simulink model "aerodynamic_model_V1_2_Wrench"  (R2025b)
settings: Solver=ode4  StartTime=0.0  StopTime=0.3  FixedStep=Ts  RelTol=1e-3
InitFcn:
  | % Run initial_main.m first to load Ad,As,Tq_prop,Tq_mass,...
values from neighbouring files (symbols this model uses):
  alpha_du0_v_tail_L = trim_aero_ic.v_tail_L.alpha_du0    [initial_main_V1_1.m]
  alpha_du0_v_tail_R = trim_aero_ic.v_tail_R.alpha_du0    [initial_main_V1_1.m]
  alpha_du0_wing_L = trim_aero_ic.wing_L.alpha_du0    [initial_main_V1_1.m]
  alpha_du0_wing_R = trim_aero_ic.wing_R.alpha_du0    [initial_main_V1_1.m]
  As = sys_sd.A    [initial_main_V1_1.m]
  BladePitch_deg = 34    [initial_main_V1_1.m]
  Bs = sys_sd.B    [initial_main_V1_1.m]
  Cs = sys_sd.C    [initial_main_V1_1.m]
  ctrl_delta_lim_deg = strips.delta_lim_deg    [initial_main_V1_1.m]
  ctrl_map_aileron_L = aero.wing_L.map_aileron(:)    [initial_main_V1_1.m]
  ctrl_map_aileron_R = aero.wing_R.map_aileron(:)    [initial_main_V1_1.m]
  ctrl_map_tail_L = aero.v_tail_L.map_tail(:)    [initial_main_V1_1.m]
  ctrl_map_tail_R = aero.v_tail_R.map_tail(:)    [initial_main_V1_1.m]
  Ds = sys_sd.D    [initial_main_V1_1.m]
  I_cg_b = R_sb * I_cg_m * R_sb.'    [aeroelastic.m]    (also in initial_main_V1_1.m = grav.I_cg_b)
  I_cg_b_inv = R_sb * I_cg_m_inv * R_sb.'    [aeroelastic.m]    (also in initial_main_V1_1.m = grav.I_cg_b_inv)
  m_node = zeros(n_id, 1)    [aeroelastic.m]    (also in generate_pullup_load_cloud.m = evalin('base', 'm_node(:)'); initial_main_V1_1.m = nodal.m_node)
  m_total_kg = evalin('base', 'm_total_kg')    [generate_pullup_load_cloud.m]    (also in initial_main_V1_1.m = grav.m_total_kg)
  n_modes = size(Phi, 2)    [aeroelastic.m]    (also in initial_main_V1_1.m = n_rigid + n_elastic)
  ones_1_tail = ones(1, size(r_cg2ac_b_v_tail_L, 2))    [initial_main_V1_1.m]
  ones_1_wing = ones(1, size(r_cg2ac_b_wing_L, 2))    [initial_main_V1_1.m]
  Phi = evalin('base', 'Phi')    [generate_pullup_load_cloud.m]    (also in initial_main_V1_1.m = strips.Phi)
  polar_alpha_deg = polar.alpha_deg(:).'    [initial_main_V1_1.m]
  polar_CD = polar.CD(:).'    [initial_main_V1_1.m]
  polar_CDp = polar.CDp(:).'    [initial_main_V1_1.m]
  polar_CL = polar.CL(:).'    [initial_main_V1_1.m]
  polar_CM = polar.CM(:).'    [initial_main_V1_1.m]
  r_cg2ac_b_v_tail_L = R_sb * aero.v_tail_L.r_ac_s    [initial_main_V1_1.m]
  r_cg2ac_b_v_tail_R = R_sb * aero.v_tail_R.r_ac_s    [initial_main_V1_1.m]
  r_cg2ac_b_wing_L = R_sb * aero.wing_L.r_ac_s    [initial_main_V1_1.m]
  r_cg2ac_b_wing_R = R_sb * aero.wing_R.r_ac_s    [initial_main_V1_1.m]
  r_cg2kink_b = eng.r_cg2kink_b    [initial_main_V1_1.m]
  r_cg2node_b = aeroelastic.node_arms(nodes, 'R_sb', R_sb).r_cg2node_b    [initial_main_V1_1.m]
  surface_nodes = aeroelastic.surface_load_nodes(nodes)    [initial_main_V1_1.m]
  T_aero2W = aeroelastic.wing_aileron_to_W(strips).T    [initial_main_V1_1.m]
  T_prop2W = load_maps.T_prop2W    [initial_main_V1_1.m]
  Tq_mass = load_maps.Tq_mass    [initial_main_V1_1.m]
  trim_Attitude_rad0 = trim_default.Attitude_rad0    [initial_main_V1_1.m]
  trim_Omega_b0 = trim_default.Omega_b0    [initial_main_V1_1.m]
  trim_Position0 = trim_default.Position0    [initial_main_V1_1.m]
  trim_Velocity_b0 = trim_default.Velocity_b0    [initial_main_V1_1.m]
  Ts = 0.001    [initial_main_V1_1.m]
  U = 55    [initial_main_V1_1.m]
  v_tail_cant_rad = deg2rad(v_tail_cant_deg)    [initial_main_V1_1.m]
  W_mass_g = grav.W_mass    [initial_main_V1_1.m]
  x0_structure = trim_default.x0_structure    [initial_main_V1_1.m]
  x0_wagner_v_tail_L = trim_aero_ic.v_tail_L.x0_wagner    [initial_main_V1_1.m]
  x0_wagner_v_tail_R = trim_aero_ic.v_tail_R.x0_wagner    [initial_main_V1_1.m]
  x0_wagner_wing_L = trim_aero_ic.wing_L.x0_wagner    [initial_main_V1_1.m]
  x0_wagner_wing_R = trim_aero_ic.wing_R.x0_wagner    [initial_main_V1_1.m]
undefined symbols (not defined in the file or in its folder): Ad_v_tail_L, Ad_v_tail_R, Ad_wing_L, Ad_wing_R, Bd_v_tail_L, Bd_v_tail_R, Bd_wing_L, Bd_wing_R, c_over_2U_v_tail_L, c_over_2U_v_tail_R, c_over_2U_wing_L, c_over_2U_wing_R, Cd_v_tail_L, Cd_v_tail_R, Cd_wing_L, Cd_wing_R, Dd_v_tail_L, Dd_v_tail_R, Dd_wing_L, Dd_wing_R, G_du_v_tail_L, G_du_v_tail_R, G_du_wing_L, G_du_wing_R, polar_aileron_alpha_deg, polar_aileron_dCD, polar_aileron_dCL, polar_aileron_dCM, polar_aileron_delta_deg, polar_ruddervator_alpha_deg, polar_ruddervator_dCD, polar_ruddervator_dCL, polar_ruddervator_dCM, polar_ruddervator_delta_deg, qS_strip_v_tail_L, qS_strip_v_tail_R, qS_strip_wing_L, qS_strip_wing_R, qSc_strip_v_tail_L, qSc_strip_v_tail_R, qSc_strip_wing_L, qSc_strip_wing_R, T_m2b_v_tail_L, T_m2b_v_tail_R, T_m2b_wing_L, T_m2b_wing_R, T_m2h_v_tail_L, T_m2h_v_tail_R, T_m2h_wing_L, T_m2h_wing_R, Tq_CM_v_tail_L, Tq_CM_v_tail_R, Tq_CM_wing_L, Tq_CM_wing_R, Tq_D_v_tail_L, Tq_D_v_tail_R, Tq_D_wing_L, Tq_D_wing_R, Tq_v_tail_L, Tq_v_tail_R ... (+2)
libraries: Prop_gryo x12, matrix_library x2
(part 6 of 6)

== matlab function aerodynamic_model_V1_2_Wrench/Load Estimator/Engine_station1/Subsystem7/MATLAB Function1 ==
  data: F input; F_b output; M input; r input; M_b output; p input
function [F_b, M_b] = wrench_to_cg(F, M, r,p) %#codegen
%WRENCH_TO_CG  节点力/力矩合到质心
%
%  [F_cg, M_cg] = wrench_to_cg(F, M, r)
%
%  F, M, r  3×n  每列一个节点，必须同一坐标系
%            r 用 r_cg2node_m（结构）或 r_cg2node_b（机体）
%  F_cg     3×1  Σ F
%  M_cg     3×1  Σ (r × F + M)
%
%  不要把 6 维扳手整段叉乘。力只求和；力矩才是 r×F 再加节点力矩。
n=size(r,2);
for i=1:n
    r(:,i)=r(:,i)-p;
end
    F_b = sum(F, 2);
    M_b = sum(cross3n(r, F) + M, 2);
end

== matlab function aerodynamic_model_V1_2_Wrench/Load Estimator/Engine_station1/Subsystem7/MATLAB Function2 ==
  data: F input; F_b output; M input; r input; M_b output; p input
function [F_b, M_b] = wrench_to_cg(F, M, r,p) %#codegen
%WRENCH_TO_CG  节点力/力矩合到质心
%
%  [F_cg, M_cg] = wrench_to_cg(F, M, r)
%
%  F, M, r  3×n  每列一个节点，必须同一坐标系
%            r 用 r_cg2node_m（结构）或 r_cg2node_b（机体）
%  F_cg     3×1  Σ F
%  M_cg     3×1  Σ (r × F + M)
%
%  不要把 6 维扳手整段叉乘。力只求和；力矩才是 r×F 再加节点力矩。
n=size(r,2);
for i=1:n
    r(:,i)=r(:,i)-p;
end
    F_b = sum(F, 2);
    M_b = sum(cross3n(r, F) + M, 2);
end

== matlab function aerodynamic_model_V1_2_Wrench/Load Estimator/Engine_station1/Subsystem7/MATLAB Function3 ==
  data: F input; F_b output; M input; r input; M_b output; p input
function [F_b, M_b] = wrench_to_cg(F, M, r,p) %#codegen
%WRENCH_TO_CG  节点力/力矩合到质心
%
%  [F_cg, M_cg] = wrench_to_cg(F, M, r)
%
%  F, M, r  3×n  每列一个节点，必须同一坐标系
%            r 用 r_cg2node_m（结构）或 r_cg2node_b（机体）
%  F_cg     3×1  Σ F
%  M_cg     3×1  Σ (r × F + M)
%
%  不要把 6 维扳手整段叉乘。力只求和；力矩才是 r×F 再加节点力矩。
n=size(r,2);
for i=1:n
    r(:,i)=r(:,i)-p;
end
    F_b = sum(F, 2);
    M_b = sum(cross3n(r, F) + M, 2);
end

== matlab function aerodynamic_model_V1_2_Wrench/Load Estimator/Structural_Station_Section1/MATLAB Function1 ==
  data: F input; F_b output; M input; r input; M_b output; p input
function [F_b, M_b] = wrench_to_cg(F, M, r,p) %#codegen
%WRENCH_TO_CG  节点力/力矩合到质心
%
%  [F_cg, M_cg] = wrench_to_cg(F, M, r)
%
%  F, M, r  3×n  每列一个节点，必须同一坐标系
%            r 用 r_cg2node_m（结构）或 r_cg2node_b（机体）
%  F_cg     3×1  Σ F
%  M_cg     3×1  Σ (r × F + M)
%
%  不要把 6 维扳手整段叉乘。力只求和；力矩才是 r×F 再加节点力矩。
n=size(r,2);
for i=1:n
    r(:,i)=r(:,i)-p;
end
    F_b = sum(F, 2);
    M_b = sum(cross3n(r, F) + M, 2);
end

== matlab function aerodynamic_model_V1_2_Wrench/Load Estimator/Structural_Station_Section1/MATLAB Function2 ==
  data: F input; F_b output; M input; r input; M_b output; p input
function [F_b, M_b] = wrench_to_cg(F, M, r,p) %#codegen
%WRENCH_TO_CG  节点力/力矩合到质心
%
%  [F_cg, M_cg] = wrench_to_cg(F, M, r)
%
%  F, M, r  3×n  每列一个节点，必须同一坐标系
%            r 用 r_cg2node_m（结构）或 r_cg2node_b（机体）
%  F_cg     3×1  Σ F
%  M_cg     3×1  Σ (r × F + M)
%
%  不要把 6 维扳手整段叉乘。力只求和；力矩才是 r×F 再加节点力矩。
n=size(r,2);
for i=1:n
    r(:,i)=r(:,i)-p;
end
    F_b = sum(F, 2);
    M_b = sum(cross3n(r, F) + M, 2);
end

== matlab function aerodynamic_model_V1_2_Wrench/Load Estimator/Structural_Station_Section1/MATLAB Function3 ==
  data: F input; F_b output; M input; r input; M_b output; p input
function [F_b, M_b] = wrench_to_cg(F, M, r,p) %#codegen
%WRENCH_TO_CG  节点力/力矩合到质心
%
%  [F_cg, M_cg] = wrench_to_cg(F, M, r)
%
%  F, M, r  3×n  每列一个节点，必须同一坐标系
%            r 用 r_cg2node_m（结构）或 r_cg2node_b（机体）
%  F_cg     3×1  Σ F
%  M_cg     3×1  Σ (r × F + M)
%
%  不要把 6 维扳手整段叉乘。力只求和；力矩才是 r×F 再加节点力矩。
n=size(r,2);
for i=1:n
    r(:,i)=r(:,i)-p;
end
    F_b = sum(F, 2);
    M_b = sum(cross3n(r, F) + M, 2);
end

== matlab function aerodynamic_model_V1_2_Wrench/Load Estimator/Wing_Section1/MATLAB Function1 ==
  data: F input; F_b output; M input; r input; p input; M_b output
function [F_b, M_b] = wrench_to_cg(F, M, r,p) %#codegen
%WRENCH_TO_CG  节点力/力矩合到质心
%
%  [F_cg, M_cg] = wrench_to_cg(F, M, r)
%
%  F, M, r  3×n  每列一个节点，必须同一坐标系
%            r 用 r_cg2node_m（结构）或 r_cg2node_b（机体）
%  F_cg     3×1  Σ F
%  M_cg     3×1  Σ (r × F + M)
%
%  不要把 6 维扳手整段叉乘。力只求和；力矩才是 r×F 再加节点力矩。
n=size(r,2);
for i=1:n
    r(:,i)=r(:,i)-p;
end
    F_b = sum(F, 2);
    M_b = sum(cross3n(r, F) + M, 2);
end

== matlab function aerodynamic_model_V1_2_Wrench/Load Estimator/Structural_Station_Section/MATLAB Function1 ==
  data: F input; F_b output; M input; r input; M_b output; p input
function [F_b, M_b] = wrench_to_cg(F, M, r,p) %#codegen
%WRENCH_TO_CG  节点力/力矩合到质心
%
%  [F_cg, M_cg] = wrench_to_cg(F, M, r)
%
%  F, M, r  3×n  每列一个节点，必须同一坐标系
%            r 用 r_cg2node_m（结构）或 r_cg2node_b（机体）
%  F_cg     3×1  Σ F
%  M_cg     3×1  Σ (r × F + M)
%
%  不要把 6 维扳手整段叉乘。力只求和；力矩才是 r×F 再加节点力矩。
n=size(r,2);
for i=1:n
    r(:,i)=r(:,i)-p;
end
    F_b = sum(F, 2);
    M_b = sum(cross3n(r, F) + M, 2);
end

== matlab function aerodynamic_model_V1_2_Wrench/Load Estimator/Wing_Section1/MATLAB Function2 ==
  data: F input; F_b output; M input; r input; M_b output; p input
function [F_b, M_b] = wrench_to_cg(F, M, r,p) %#codegen
%WRENCH_TO_CG  节点力/力矩合到质心
%
%  [F_cg, M_cg] = wrench_to_cg(F, M, r)
%
%  F, M, r  3×n  每列一个节点，必须同一坐标系
%            r 用 r_cg2node_m（结构）或 r_cg2node_b（机体）
%  F_cg     3×1  Σ F
%  M_cg     3×1  Σ (r × F + M)
%
%  不要把 6 维扳手整段叉乘。力只求和；力矩才是 r×F 再加节点力矩。
n=size(r,2);
for i=1:n
    r(:,i)=r(:,i)-p;
end
    F_b = sum(F, 2);
    M_b = sum(cross3n(r, F) + M, 2);
end

== matlab function aerodynamic_model_V1_2_Wrench/Load Estimator/Wing_Section1/MATLAB Function3 ==
  data: F input; F_b output; M input; r input; M_b output; p input
function [F_b, M_b] = wrench_to_cg(F, M, r,p) %#codegen
%WRENCH_TO_CG  节点力/力矩合到质心
%
%  [F_cg, M_cg] = wrench_to_cg(F, M, r)
%
%  F, M, r  3×n  每列一个节点，必须同一坐标系
%            r 用 r_cg2node_m（结构）或 r_cg2node_b（机体）
%  F_cg     3×1  Σ F
%  M_cg     3×1  Σ (r × F + M)
%
%  不要把 6 维扳手整段叉乘。力只求和；力矩才是 r×F 再加节点力矩。
n=size(r,2);
for i=1:n
    r(:,i)=r(:,i)-p;
end
    F_b = sum(F, 2);
    M_b = sum(cross3n(r, F) + M, 2);
end

== matlab function aerodynamic_model_V1_2_Wrench/Load Estimator/Wing_Section1/MATLAB Function4 ==
  data: F input; F_b output; M input; r input; M_b output; p input
function [F_b, M_b] = wrench_to_cg(F, M, r,p) %#codegen
%WRENCH_TO_CG  节点力/力矩合到质心
%
%  [F_cg, M_cg] = wrench_to_cg(F, M, r)
%
%  F, M, r  3×n  每列一个节点，必须同一坐标系
%            r 用 r_cg2node_m（结构）或 r_cg2node_b（机体）
%  F_cg     3×1  Σ F
%  M_cg     3×1  Σ (r × F + M)
%
%  不要把 6 维扳手整段叉乘。力只求和；力矩才是 r×F 再加节点力矩。
n=size(r,2);
for i=1:n
    r(:,i)=r(:,i)-p;
end
    F_b = sum(F, 2);
    M_b = sum(cross3n(r, F) + M, 2);
end

== matlab function aerodynamic_model_V1_2_Wrench/Strip Aerodynamics/Local_Alphas/MATLAB Function3 ==
  data: V input; alpha output; beta output
function [alpha, beta] = fcn(V)
[alpha, beta] = strip_aero_angles(V);
end

== matlab function aerodynamic_model_V1_2_Wrench/Load Estimator/Structural_Station_Section/MATLAB Function2 ==
  data: F input; F_b output; M input; r input; M_b output; p input
function [F_b, M_b] = wrench_to_cg(F, M, r,p) %#codegen
%WRENCH_TO_CG  节点力/力矩合到质心
%
%  [F_cg, M_cg] = wrench_to_cg(F, M, r)
%
%  F, M, r  3×n  每列一个节点，必须同一坐标系
%            r 用 r_cg2node_m（结构）或 r_cg2node_b（机体）
%  F_cg     3×1  Σ F
%  M_cg     3×1  Σ (r × F + M)
%
%  不要把 6 维扳手整段叉乘。力只求和；力矩才是 r×F 再加节点力矩。
n=size(r,2);
for i=1:n
    r(:,i)=r(:,i)-p;
end
    F_b = sum(F, 2);
    M_b = sum(cross3n(r, F) + M, 2);
end
